simulink model "Full_Car_Model"  (R2023b)
settings: Solver=FixedStepAuto  StartTime=0.0  StopTime=t_end_sim  FixedStep=Ts_sim  RelTol=1e-3
values from neighbouring files (symbols this model uses):
  a_b_ref_sat = [ zeros(1,10) ... (first row only)    [A1_Init.m]    (also in C1_MonteCarloAnalysis.m)
  adaptive = 3    [A1_Init.m]    (also in C1_MonteCarloAnalysis.m = 1)
  data = A2_Full_car_model_parameters_4onBoard()    [A1_Init.m]    (also in C1_MonteCarloAnalysis.m)
  Ft_demand_F = [zeros(1,601) 200*ones(1,2400)]./data.R_F    [A1_Init.m]    (also in C1_MonteCarloAnalysis.m)
  Ft_demand_R = [zeros(1,(601-length(l_discr)))              200*ones(1,(2400+length(l_discr)))]./data.R_R    [A1_Init.m]    (also in C1_MonteCarloAnalysis.m)
  handmade_front = strcat(currentPath,'\Road_profiles\height_crg_files\','handmade_step_3cm_singlefunctions.crg')    [A1_Init.m]    (also in C1_MonteCarloAnalysis.m)
  handmade_mu_front = strcat(currentPath,'\Road_profiles\friction_crg_files\','handmade_fric_step_01_singlefunctions.crg')    [A1_Init.m]    (also in C1_MonteCarloAnalysis.m)
  handmade_mu_rear = handmade_mu_front    [A1_Init.m]    (also in C1_MonteCarloAnalysis.m)
  handmade_rear = handmade_front    [A1_Init.m]    (also in C1_MonteCarloAnalysis.m)
  LowLim_Q1 = -10    [A1_Init.m]    (also in C1_MonteCarloAnalysis.m)
  M = N    (= 10)    [A1_Init.m]    (also in C1_MonteCarloAnalysis.m)
  mu_distance = test_distance    [A1_Init.m]    (also in C1_MonteCarloAnalysis.m)
  mu_road = [ones(1,1001), 0.1*ones(1,2000)]    [A1_Init.m]    (also in C1_MonteCarloAnalysis.m)
  N = 10    [A1_Init.m]    (also in C1_MonteCarloAnalysis.m)
  N_iter = 3    [A1_Init.m]    (also in C1_MonteCarloAnalysis.m)
  omega_ini_F_L = x_u_dot_ini_F_L/data.R_F    [A1_Init.m]    (also in C1_MonteCarloAnalysis.m)
  omega_ini_F_R = x_u_dot_ini_R_R/data.R_F    [A1_Init.m]    (also in C1_MonteCarloAnalysis.m)
  omega_ini_R_L = x_u_dot_ini_R_L/data.R_R +2.483*1e-6    [A1_Init.m]    (also in C1_MonteCarloAnalysis.m)
  omega_ini_R_R = x_u_dot_ini_R_R/data.R_R+2.483*1e-6    [A1_Init.m]    (also in C1_MonteCarloAnalysis.m)
  passive = 2    [A1_Init.m]    (also in C1_MonteCarloAnalysis.m)
  Pitch = 0    [A1_Init.m]    (also in C1_MonteCarloAnalysis.m)
  Pitch_dot = 0    [A1_Init.m]    (also in C1_MonteCarloAnalysis.m)
  preview = 2    [A1_Init.m]    (also in C1_MonteCarloAnalysis.m)
  Q1 = 1e6    (= 1000000)    [A1_Init.m]    (also in C1_MonteCarloAnalysis.m)
  Q1_sat = 0    [A1_Init.m]    (also in C1_MonteCarloAnalysis.m)
  Q2 = 1e5    (= 100000)    [A1_Init.m]    (also in C1_MonteCarloAnalysis.m)
  QN1 = 0    [A1_Init.m]    (also in C1_MonteCarloAnalysis.m)
  QN2 = 0    [A1_Init.m]    (also in C1_MonteCarloAnalysis.m)
  R1 = 1e10    (= 10000000000)    [A1_Init.m]    (also in C1_MonteCarloAnalysis.m)
  r1_h0 = 0.99    [A1_Init.m]    (also in C1_MonteCarloAnalysis.m)
  r1_k = 1000    [A1_Init.m]    (also in C1_MonteCarloAnalysis.m)
  r1_max = 11    [A1_Init.m]    (also in C1_MonteCarloAnalysis.m)
  r1_min = -10    [A1_Init.m]    (also in C1_MonteCarloAnalysis.m)
  r2 = 2    [A1_Init.m]    (also in C1_MonteCarloAnalysis.m)
  R2 = 1e2    (= 100)    [A1_Init.m]    (also in C1_MonteCarloAnalysis.m)
  R2_rl = 2    [A1_Init.m]    (also in C1_MonteCarloAnalysis.m)
  road_profile = [zeros(1,801),ones(1,2200)*10*Step_selector]    [A1_Init.m]    (also in C1_MonteCarloAnalysis.m)
  T_distance = test_distance    [A1_Init.m]    (also in C1_MonteCarloAnalysis.m)
  T_hs_ini_F_L = 0    [A1_Init.m]    (also in C1_MonteCarloAnalysis.m)
  T_hs_ini_F_R = 0    [A1_Init.m]    (also in C1_MonteCarloAnalysis.m)
  T_hs_ini_R_L = 0    [A1_Init.m]    (also in C1_MonteCarloAnalysis.m)
  T_hs_ini_R_R = 0    [A1_Init.m]    (also in C1_MonteCarloAnalysis.m)
  test_distance = 0:0.01:30    [A1_Init.m]    (also in C1_MonteCarloAnalysis.m)
  theta_s_ini_F_L = 0    [A1_Init.m]    (also in C1_MonteCarloAnalysis.m)
  theta_s_ini_F_R = 0    [A1_Init.m]    (also in C1_MonteCarloAnalysis.m)
  theta_s_ini_R_L = 0    [A1_Init.m]    (also in C1_MonteCarloAnalysis.m)
  theta_s_ini_R_R = 0    [A1_Init.m]    (also in C1_MonteCarloAnalysis.m)
  theta_w_ini_F_L = -1.056*1e-2    (= -0.01056)    [A1_Init.m]    (also in C1_MonteCarloAnalysis.m)
  theta_w_ini_R_L = -1.056*1e-2    (= -0.01056)    [A1_Init.m]    (also in C1_MonteCarloAnalysis.m)
  Ts = 1e-3*[0 5 10 15 20 25 30 40 60 80 100]    [A1_Init.m]    (also in C1_MonteCarloAnalysis.m)
  w1_h0 = 0.0008    [A1_Init.m]    (also in C1_MonteCarloAnalysis.m)
  w1_k = 5000    [A1_Init.m]    (also in C1_MonteCarloAnalysis.m)
  w1_max = 9    [A1_Init.m]    (also in C1_MonteCarloAnalysis.m)
  w1_min = -10    [A1_Init.m]    (also in C1_MonteCarloAnalysis.m)
  w1_sat = 0.085    [A1_Init.m]    (also in C1_MonteCarloAnalysis.m)
  w2_h0 = 2    [A1_Init.m]    (also in C1_MonteCarloAnalysis.m)
  w2_inc = 0.05    [A1_Init.m]    (also in C1_MonteCarloAnalysis.m)
  w2_k = 10    [A1_Init.m]    (also in C1_MonteCarloAnalysis.m)
  w2_max = 5.3    [A1_Init.m]    (also in C1_MonteCarloAnalysis.m)
  w2_min = -10    [A1_Init.m]    (also in C1_MonteCarloAnalysis.m)
  Wmat_NMPC_init = [W(1,:) W(2,:) W(3,:) W(4,:)]    [A1_Init.m]    (also in C1_MonteCarloAnalysis.m)
  WNmat_NMPC_init = [WN(1,:) WN(2,:)]    [A1_Init.m]    (also in C1_MonteCarloAnalysis.m)
  X_0 = [z_b_dot_ini z_b_ini z_u_dot_ini_F_L z_u_ini_F_L x_b_dot_ini x_b_ini x_u_dot_ini_F_L x_u_ini_F_L          omega_ini_F_L theta_w_ini_F_L omega_ini_F_L theta_s_ini_F_L torque_ini_F_L]    [A1_Init.m]    (also in C1_MonteCarloAnalysis.m)
  x_b_dot_ini = speed_ini/3.6    (= 11.1111111111)    [A1_Init.m]    (also in C1_MonteCarloAnalysis.m)
  x_b_ini = data.b+pos_ini    [A1_Init.m]    (also in C1_MonteCarloAnalysis.m)
  x_u_dot_ini_F_L = speed_ini/3.6 - 1.125*1e-4    (= 11.1109986111)    [A1_Init.m]    (also in C1_MonteCarloAnalysis.m)
  x_u_dot_ini_F_R = speed_ini/3.6 - 1.125*1e-4    (= 11.1109986111)    [A1_Init.m]    (also in C1_MonteCarloAnalysis.m)
  x_u_dot_ini_R_L = speed_ini/3.6 - 1.125*1e-4    (= 11.1109986111)    [A1_Init.m]    (also in C1_MonteCarloAnalysis.m)
  x_u_dot_ini_R_R = speed_ini/3.6 - 1.125*1e-4    (= 11.1109986111)    [A1_Init.m]    (also in C1_MonteCarloAnalysis.m)
  x_u_ini_F_L = data.a+data.b+pos_ini    [A1_Init.m]    (also in C1_MonteCarloAnalysis.m)
  x_u_ini_F_R = data.a+data.b+pos_ini    [A1_Init.m]    (also in C1_MonteCarloAnalysis.m)
  x_u_ini_R_L = pos_ini    (= 0)    [A1_Init.m]    (also in C1_MonteCarloAnalysis.m)
  x_u_ini_R_R = pos_ini    (= 0)    [A1_Init.m]    (also in C1_MonteCarloAnalysis.m)
  z_b_dot_ini = 0    [A1_Init.m]    (also in C1_MonteCarloAnalysis.m)
  z_b_ini = 0    [A1_Init.m]    (also in C1_MonteCarloAnalysis.m)
  z_u_dot_ini_F_L = 0    [A1_Init.m]    (also in C1_MonteCarloAnalysis.m)
  z_u_dot_ini_F_R = 0    [A1_Init.m]    (also in C1_MonteCarloAnalysis.m)
  z_u_dot_ini_R_L = 0    [A1_Init.m]    (also in C1_MonteCarloAnalysis.m)
  z_u_dot_ini_R_R = 0    [A1_Init.m]    (also in C1_MonteCarloAnalysis.m)
  z_u_ini_F_L = 0    [A1_Init.m]    (also in C1_MonteCarloAnalysis.m)
  z_u_ini_F_R = 0    [A1_Init.m]    (also in C1_MonteCarloAnalysis.m)
  z_u_ini_R_L = 0    [A1_Init.m]    (also in C1_MonteCarloAnalysis.m)
  z_u_ini_R_R = 0    [A1_Init.m]    (also in C1_MonteCarloAnalysis.m)
undefined symbols (not defined in the file or in its folder): Delay_step, road_with_noise
libraries: mfswift_library x8, rllib x4, simulink x4
(part 5 of 7)

== system Full_Car_Model/CONTROLLER REAR RIGHT/Rule based/Subsystem ==
  Online Data : Inport
  Delay{,1..4} (5 alike) : Delay  DelayLength=10
  Delay{5..34} (30 alike) : Delay  DelayLength=1
  MATLAB Function : MATLAB Function  TreatAsAtomicUnit=on
  Mux : Mux  Inputs=5
  Mux1 : Mux  Inputs=30
  Mux2 : Mux  Inputs=2
  Rate Transition : RateTransition  OutPortSampleTime=Ts(2)
  Rate Transition1 : RateTransition  OutPortSampleTime=Ts(2)
  Selector : Selector  NumberOfDimensions=2  InputPortWidth=1  IndexOptions=Index vector (dialog),Select all  Indices=1,1  OutputSizes=1,1
  Selector1 : Selector  NumberOfDimensions=2  InputPortWidth=1  IndexOptions=Index vector (dialog),Select all  Indices=1,1  OutputSizes=1,1
  w_prev : Outport
  mu_act_prev : Outport  Port=2
  wires:
  MATLAB Function/1(w) -> Mux2/2, Selector/1, Selector1/1
  MATLAB Function/2(mu_act) -> mu_act_prev/1
  Mux1/1 -> Rate Transition1/1
  Rate Transition/1 -> MATLAB Function/1(OnlineData)
  Mux2/1 -> w_prev/1
  Delay4/1 -> Mux/1
  Delay3/1 -> Delay4/1, Mux/2
  Delay2/1 -> Delay3/1, Mux/3
  Delay1/1 -> Mux/4, Delay2/1
  Delay/1 -> Mux/5, Delay1/1
  Selector/1 -> Delay/1  "w1"
  Online Data/1 -> Rate Transition/1
  Delay5/1 -> Mux1/8, Delay10/1
  Selector1/1 -> Delay29/1  "w1"
  Delay10/1 -> Mux1/7, Delay11/1
  Delay11/1 -> Mux1/6, Delay12/1
  Delay12/1 -> Mux1/5, Delay13/1
  Delay13/1 -> Mux1/4, Delay14/1
  Delay14/1 -> Mux1/3, Delay15/1
  Delay15/1 -> Mux1/2, Delay16/1
  Delay16/1 -> Mux1/1
  Delay6/1 -> Mux1/9, Delay5/1
  Delay7/1 -> Mux1/10, Delay6/1
  Delay8/1 -> Delay7/1, Mux1/11
  Delay9/1 -> Mux1/12, Delay8/1
  Delay17/1 -> Mux1/13, Delay9/1
  Delay18/1 -> Mux1/14, Delay17/1
  Delay19/1 -> Delay18/1, Mux1/15
  Delay26/1 -> Mux1/16, Delay19/1
  Delay25/1 -> Mux1/17, Delay26/1
  Delay24/1 -> Mux1/18, Delay25/1
  Delay22/1 -> Mux1/20, Delay23/1
  Delay34/1 -> Mux1/27, Delay33/1
  Delay33/1 -> Mux1/26, Delay32/1
  Delay31/1 -> Mux1/24, Delay30/1
  Delay32/1 -> Mux1/25, Delay31/1
  Delay30/1 -> Mux1/23, Delay20/1
  Delay28/1 -> Mux1/29, Delay27/1
  Delay27/1 -> Mux1/28, Delay34/1
  Delay23/1 -> Mux1/19, Delay24/1
  Delay21/1 -> Mux1/21, Delay22/1
  Delay29/1 -> Mux1/30, Delay28/1
  Delay20/1 -> Mux1/22, Delay21/1
  Mux/1 -> Mux2/1

== system Full_Car_Model/CONTROLLER REAR RIGHT/Rule based/memory ==
  In1 : Inport
  Abs : Abs  SaturateOnIntegerOverflow=off
  Add : Sum  Inputs=-+
  Memory{,1..10,12..15,19,26..49} (40 alike) : Memory  InheritSampleTime=on
  Mux1 : Mux  Inputs=40
  Rate Transition : RateTransition  OutPortSampleTime=Ts(2)
  Out1 : Outport
  wires:
  Abs/1 -> Mux1/40, Memory49/1
  Memory49/1 -> Mux1/39, Memory19/1
  Memory19/1 -> Memory35/1, Mux1/38
  Memory47/1 -> Memory48/1, Mux1/31
  Memory42/1 -> Memory43/1, Mux1/36
  Memory44/1 -> Memory45/1, Mux1/34
  Memory43/1 -> Memory44/1, Mux1/35
  Memory33/1 -> Memory34/1, Mux1/23
  Memory46/1 -> Memory47/1, Mux1/32
  Memory32/1 -> Memory33/1, Mux1/24
  Memory38/1 -> Memory39/1, Mux1/18
  Memory48/1 -> Memory26/1, Mux1/30
  Memory45/1 -> Memory46/1, Mux1/33
  Memory30/1 -> Memory31/1, Mux1/26
  Memory26/1 -> Memory28/1, Mux1/29
  Memory37/1 -> Memory38/1, Mux1/19
  Memory29/1 -> Memory30/1, Mux1/27
  Memory31/1 -> Memory32/1, Mux1/25
  Memory27/1 -> Memory36/1, Mux1/21
  Memory28/1 -> Memory29/1, Mux1/28
  Memory34/1 -> Memory27/1, Mux1/22
  Memory40/1 -> Memory41/1, Mux1/16
  Memory41/1 -> Mux1/15, Memory1/1
  Memory39/1 -> Memory40/1, Mux1/17
  Memory35/1 -> Memory42/1, Mux1/37
  Memory36/1 -> Memory37/1, Mux1/20
  Add/1 -> Abs/1
  In1/1 -> Rate Transition/1
  Memory/1 -> Add/1
  Rate Transition/1 -> Add/2, Memory/1
  Memory14/1 -> Memory15/1, Mux1/2
  Memory12/1 -> Memory13/1, Mux1/4
  Memory15/1 -> Mux1/1
  Memory13/1 -> Memory14/1, Mux1/3
  Memory10/1 -> Mux1/5, Memory12/1
  Memory9/1 -> Memory10/1, Mux1/6
  Memory8/1 -> Memory9/1, Mux1/7
  Memory7/1 -> Memory8/1, Mux1/8
  Memory6/1 -> Memory7/1, Mux1/9
  Memory5/1 -> Memory6/1, Mux1/10
  Memory4/1 -> Mux1/11, Memory5/1
  Memory3/1 -> Memory4/1, Mux1/12
  Memory2/1 -> Mux1/13, Memory3/1
  Memory1/1 -> Memory2/1, Mux1/14
  Mux1/1 -> Out1/1

== system Full_Car_Model/PLANT MODEL WITH MF-SWIFT/4 ON-BOARD POWERTRAIN - FRONT/DIFFERENTIAL_L ==
  T_dm : Inport
  Multiply : Gain  Gain=data.i_g1_F4
  Multiply1 : Gain  Gain=data.n_g1_F4
  Multiply2 : Gain  Gain=data.i_g2_F4
  Multiply3 : Gain  Gain=data.n_g2_F4
  T_t : Outport
  wires:
  T_dm/1 -> Multiply/1
  Multiply3/1 -> T_t/1
  Multiply1/1 -> Multiply2/1
  Multiply2/1 -> Multiply3/1
  Multiply/1 -> Multiply1/1

== system Full_Car_Model/PLANT MODEL WITH MF-SWIFT/4 ON-BOARD POWERTRAIN - FRONT/DIFFERENTIAL_R ==
  T_dm : Inport
  Multiply : Gain  Gain=data.i_g1_F4
  Multiply1 : Gain  Gain=data.n_g1_F4
  Multiply2 : Gain  Gain=data.i_g2_F4
  Multiply3 : Gain  Gain=data.n_g2_F4
  T_t : Outport
  wires:
  Multiply3/1 -> T_t/1
  Multiply/1 -> Multiply1/1
  Multiply1/1 -> Multiply2/1
  Multiply2/1 -> Multiply3/1
  T_dm/1 -> Multiply/1

== system Full_Car_Model/PLANT MODEL WITH MF-SWIFT/4 ON-BOARD POWERTRAIN - FRONT/LEFT HALF SHAFT TORQUES WITH BACKLASH ==
  omega_s : Inport
  theta_s : Inport  Port=2
  theta_w : Inport  Port=3
  omega_w : Inport  Port=4
  Add1 : Sum  Inputs=+-
  Add2 : Sum  Inputs=+-
  Add{3..5,7} (4 alike) : Sum
  Add6 : Sum  Inputs=+-
  Constant : Constant  Value=data.backlash_F4
  Constant1 : Constant  Value=data.backlash_F4
  Constant2 : Constant  Value=data.backlash_F4
  MATLAB Function2 : MATLAB Function  TreatAsAtomicUnit=on
  MATLAB Function3 : MATLAB Function  TreatAsAtomicUnit=on
  Multiply1 : Gain  Gain=data.k_hs_F4
  Multiply2 : Gain  Gain=data.k_hs_F4
  Multiply3 : Gain  Gain=data.b_hs_F4
  Product{1..4} (4 alike) : Product
  T_hs : Outport
  wires:
  [delta_omega_F_L] -> Multiply3/1
  [delta_theta_F_L] -> MATLAB Function3/1(delta_theta)
  Add1/1 -> [delta_omega_F_L]  "delta_omega"
  [delta_theta_F_L] -> Add6/1
  [delta_theta_F_L] -> Add7/1
  [delta_theta_F_L] -> MATLAB Function2/1(delta_theta)
  Add2/1 -> [delta_theta_F_L]  "delta_theta"
  Multiply3/1 -> Product4/1, Product3/1  "fc"
  Add6/1 -> Multiply1/1
  Constant1/1 -> Add6/2
  Multiply1/1 -> Product1/1  "fb"
  Constant/1 -> Add7/2
  Add7/1 -> Multiply2/1
  Product1/1 -> Add4/2
  Product2/1 -> Add4/1
  Product3/1 -> Add3/1
  Product4/1 -> Add3/2
  Add3/1 -> Add5/2  "T_hs_D"
  Add4/1 -> Add5/1  "T_hs_S"
  MATLAB Function3/1(f2) -> Product4/2, Product1/2  "f2"
  MATLAB Function2/1(f1) -> Product3/2, Product2/2  "f1"
  Multiply2/1 -> Product2/1  "fa"
  omega_s/1 -> Add1/1
  omega_w/1 -> Add1/2
  theta_w/1 -> Add2/2
  theta_s/1 -> Add2/1
  Add5/1 -> T_hs/1
  Constant2/1 -> MATLAB Function2/2(backlash_F4), MATLAB Function3/2(backlash_F4)

== system Full_Car_Model/PLANT MODEL WITH MF-SWIFT/4 ON-BOARD POWERTRAIN - FRONT/RIGHT HALF SHAFT TORQUES WITH BACKLASH ==
  omega_s : Inport
  theta_s : Inport  Port=2
  theta_w : Inport  Port=3
  omega_w : Inport  Port=4
  Add1 : Sum  Inputs=+-
  Add2 : Sum  Inputs=+-
  Add{3..5,7} (4 alike) : Sum
  Add6 : Sum  Inputs=+-
  Constant : Constant  Value=data.backlash_F4
  Constant1 : Constant  Value=data.backlash_F4
  Constant2 : Constant  Value=data.backlash_F4
  MATLAB Function2 : MATLAB Function  TreatAsAtomicUnit=on
  MATLAB Function3 : MATLAB Function  TreatAsAtomicUnit=on
  Multiply1 : Gain  Gain=data.k_hs_F4
  Multiply2 : Gain  Gain=data.k_hs_F4
  Multiply3 : Gain  Gain=data.b_hs_F4
  Product{1..4} (4 alike) : Product
  T_hs : Outport
  wires:
  Add5/1 -> T_hs/1
  theta_s/1 -> Add2/1
  theta_w/1 -> Add2/2
  omega_w/1 -> Add1/2
  omega_s/1 -> Add1/1
  Multiply2/1 -> Product2/1  "fa"
  MATLAB Function2/1(f1) -> Product3/2, Product2/2  "f1"
  MATLAB Function3/1(f2) -> Product1/2, Product4/2  "f2"
  Add4/1 -> Add5/1  "T_hs_S"
  Add3/1 -> Add5/2  "T_hs_D"
  Product4/1 -> Add3/2
  Product3/1 -> Add3/1
  Product2/1 -> Add4/1
  Product1/1 -> Add4/2
  Add7/1 -> Multiply2/1
  Constant/1 -> Add7/2
  Multiply1/1 -> Product1/1  "fb"
  Constant1/1 -> Add6/2
  Add6/1 -> Multiply1/1
  Multiply3/1 -> Product3/1, Product4/1  "fc"
  Add2/1 -> [delta_theta_F_R]  "delta_theta"
  [delta_theta_F_R] -> MATLAB Function2/1(delta_theta)
  [delta_theta_F_R] -> Add7/1
  [delta_theta_F_R] -> Add6/1
  Add1/1 -> [delta_omega_F_R]  "delta_omega"
  [delta_theta_F_R] -> MATLAB Function3/1(delta_theta)
  [delta_omega_F_R] -> Multiply3/1
  Constant2/1 -> MATLAB Function3/2(backlash_F4), MATLAB Function2/2(backlash_F4)

== system Full_Car_Model/PLANT MODEL WITH MF-SWIFT/4 ON-BOARD POWERTRAIN - REAR/DIFFERENTIAL_L ==
  T_dm : Inport
  Multiply : Gain  Gain=data.i_g1_R4
  Multiply1 : Gain  Gain=data.n_g1_R4
  Multiply2 : Gain  Gain=data.i_g2_R4
  Multiply3 : Gain  Gain=data.n_g2_R4
  T_t : Outport
  wires:
  T_dm/1 -> Multiply/1
  Multiply3/1 -> T_t/1
  Multiply1/1 -> Multiply2/1
  Multiply2/1 -> Multiply3/1
  Multiply/1 -> Multiply1/1

== system Full_Car_Model/PLANT MODEL WITH MF-SWIFT/4 ON-BOARD POWERTRAIN - REAR/DIFFERENTIAL_R ==
  T_dm : Inport
  Multiply : Gain  Gain=data.i_g1_R4
  Multiply1 : Gain  Gain=data.n_g1_R4
  Multiply2 : Gain  Gain=data.i_g2_R4
  Multiply3 : Gain  Gain=data.n_g2_R4
  T_t : Outport
  wires:
  Multiply/1 -> Multiply1/1
  Multiply2/1 -> Multiply3/1
  Multiply1/1 -> Multiply2/1
  Multiply3/1 -> T_t/1
  T_dm/1 -> Multiply/1

== system Full_Car_Model/PLANT MODEL WITH MF-SWIFT/4 ON-BOARD POWERTRAIN - REAR/LEFT HALF SHAFT TORQUES WITH BACKLASH ==
  omega_s : Inport
  theta_s : Inport  Port=2
  theta_w : Inport  Port=3
  omega_w : Inport  Port=4
  Add1 : Sum  Inputs=+-
  Add2 : Sum  Inputs=+-
  Add{3..5,7} (4 alike) : Sum
  Add6 : Sum  Inputs=+-
  Constant : Constant  Value=data.backlash_R4
  Constant1 : Constant  Value=data.backlash_R4
  Constant2 : Constant  Value=data.backlash_R4
  MATLAB Function2 : MATLAB Function  TreatAsAtomicUnit=on
  MATLAB Function3 : MATLAB Function  TreatAsAtomicUnit=on
  Multiply1 : Gain  Gain=data.k_hs_R4
  Multiply2 : Gain  Gain=data.k_hs_R4
  Multiply3 : Gain  Gain=data.b_hs_R4
  Product{1..4} (4 alike) : Product
  T_hs : Outport
  wires:
  [delta_omega_R_L] -> Multiply3/1
  [delta_theta_R_L] -> MATLAB Function3/1(delta_theta)
  Add1/1 -> [delta_omega_R_L]  "delta_omega"
  [delta_theta_R_L] -> Add6/1
  [delta_theta_R_L] -> Add7/1
  [delta_theta_R_L] -> MATLAB Function2/1(delta_theta)
  Add2/1 -> [delta_theta_R_L]  "delta_theta"
  Multiply3/1 -> Product4/1, Product3/1  "fc"
  Add6/1 -> Multiply1/1
  Constant1/1 -> Add6/2
  Multiply1/1 -> Product1/1  "fb"
  Constant/1 -> Add7/2
  Add7/1 -> Multiply2/1
  Product1/1 -> Add4/2
  Product2/1 -> Add4/1
  Product3/1 -> Add3/1
  Product4/1 -> Add3/2
  Add3/1 -> Add5/2  "T_hs_D"
  Add4/1 -> Add5/1  "T_hs_S"
  MATLAB Function3/1(f2) -> Product4/2, Product1/2  "f2"
  MATLAB Function2/1(f1) -> Product3/2, Product2/2  "f1"
  Multiply2/1 -> Product2/1  "fa"
  omega_s/1 -> Add1/1
  omega_w/1 -> Add1/2
  theta_w/1 -> Add2/2
  theta_s/1 -> Add2/1
  Add5/1 -> T_hs/1
  Constant2/1 -> MATLAB Function3/2(backlash_R4), MATLAB Function2/2(backlash_R4)

== system Full_Car_Model/PLANT MODEL WITH MF-SWIFT/4 ON-BOARD POWERTRAIN - REAR/RIGHT HALF SHAFT TORQUES WITH BACKLASH ==
  omega_s : Inport
  theta_s : Inport  Port=2
  theta_w : Inport  Port=3
  omega_w : Inport  Port=4
  Add1 : Sum  Inputs=+-
  Add2 : Sum  Inputs=+-
  Add{3..5,7} (4 alike) : Sum
  Add6 : Sum  Inputs=+-
  Constant : Constant  Value=data.backlash_R4
  Constant1 : Constant  Value=data.backlash_R4
  Constant2 : Constant  Value=data.backlash_R4
  MATLAB Function2 : MATLAB Function  TreatAsAtomicUnit=on
  MATLAB Function3 : MATLAB Function  TreatAsAtomicUnit=on
  Multiply1 : Gain  Gain=data.k_hs_R4
  Multiply2 : Gain  Gain=data.k_hs_R4
  Multiply3 : Gain  Gain=data.b_hs_R4
  Product{1..4} (4 alike) : Product
  T_hs : Outport
  wires:
  Add5/1 -> T_hs/1
  theta_s/1 -> Add2/1
  theta_w/1 -> Add2/2
  omega_w/1 -> Add1/2
  omega_s/1 -> Add1/1
  Multiply2/1 -> Product2/1  "fa"
  MATLAB Function2/1(f1) -> Product3/2, Product2/2  "f1"
  MATLAB Function3/1(f2) -> Product1/2, Product4/2  "f2"
  Add4/1 -> Add5/1  "T_hs_S"
  Add3/1 -> Add5/2  "T_hs_D"
  Product4/1 -> Add3/2
  Product3/1 -> Add3/1
  Product2/1 -> Add4/1
  Product1/1 -> Add4/2
  Add7/1 -> Multiply2/1
  Constant/1 -> Add7/2
  Multiply1/1 -> Product1/1  "fb"
  Constant1/1 -> Add6/2
  Add6/1 -> Multiply1/1
  Multiply3/1 -> Product3/1, Product4/1  "fc"
  Add2/1 -> [delta_theta_R_R]  "delta_theta"
  [delta_theta_R_R] -> MATLAB Function2/1(delta_theta)
  [delta_theta_R_R] -> Add7/1
  [delta_theta_R_R] -> Add6/1
  Add1/1 -> [delta_omega_R_R]  "delta_omega"
  [delta_theta_R_R] -> MATLAB Function3/1(delta_theta)
  [delta_omega_R_R] -> Multiply3/1
  Constant2/1 -> MATLAB Function3/2(backlash_R4), MATLAB Function2/2(backlash_R4)

== system Full_Car_Model/PLANT MODEL WITH MF-SWIFT/FRONT LEFT WHEEL/Subsystem ==
  speed : Inport
  Bus Selector : BusSelector  OutputSignals=States.x_u_dot_F_L,States.z_u_dot_F_L
  Constant : Constant  Value=0
  Mux : Mux  Inputs=3
  Velocity : Outport  VectorParamsAs1DForOutWhenUnconnected=off
  wires:
  Bus Selector/2 -> Mux/3  "<z_u_dot_F_L>"
  Bus Selector/1 -> Mux/1  "<x_u_dot_F_L>"
  speed/1 -> Bus Selector/1
  Mux/1 -> Velocity/1
  Constant/1 -> Mux/2  "No lateral component"

== system Full_Car_Model/PLANT MODEL WITH MF-SWIFT/FRONT LEFT WHEEL/Subsystem1 ==
  Angular Speed : Inport
  Constant1 : Constant  Value=0
  Constant2 : Constant  Value=0
  Constant3 : Constant  Value=0
  Mux : Mux  Inputs=3
  Terminator : Terminator
  AngularVelocity : Outport  VectorParamsAs1DForOutWhenUnconnected=off
  wires:
  Constant3/1 -> Mux/2
  Constant1/1 -> Mux/3
  Constant2/1 -> Mux/1
  Angular Speed/1 -> Terminator/1
  Mux/1 -> AngularVelocity/1

== system Full_Car_Model/PLANT MODEL WITH MF-SWIFT/FRONT LEFT WHEEL/Subsystem6 ==
  time : Inport
  gain : Inport  Port=2
  Demux : Demux  Outputs=9
  Multiply : Product  Inputs=**
  Mux : Mux  Inputs=20
  Step : Step  After=0.02  SampleTime=0
  Terminator : Terminator
  ground{,1..7} (8 alike) : Ground
  rotation matrix : Constant  Value=[1 0 0 0 1 0 0 0 1]
  surface friction in lateral direction : Constant
  surface friction in longitudinall direction : Constant
  Road : Outport  VectorParamsAs1DForOutWhenUnconnected=off
  wires:
  Multiply/1 -> Mux/3
  Step/1 -> Multiply/1
  gain/1 -> Multiply/2
  time/1 -> Terminator/1
  Demux/9 -> Mux/12
  Demux/8 -> Mux/11
  Demux/7 -> Mux/10
  Demux/6 -> Mux/9
  Demux/5 -> Mux/8
  Demux/4 -> Mux/7
  Demux/3 -> Mux/6
  Demux/2 -> Mux/5
  Demux/1 -> Mux/4
  rotation matrix/1 -> Demux/1
  surface friction in lateral direction/1 -> Mux/20
  surface friction in longitudinall direction/1 -> Mux/19
  ground7/1 -> Mux/18
  ground6/1 -> Mux/17
  ground5/1 -> Mux/16
  ground4/1 -> Mux/15
  ground3/1 -> Mux/14
  ground2/1 -> Mux/13
  ground1/1 -> Mux/2
  ground/1 -> Mux/1
  Mux/1 -> Road/1

== system Full_Car_Model/PLANT MODEL WITH MF-SWIFT/FRONT RIGHT WHEEL/Subsystem ==
  speed : Inport
  Bus Selector : BusSelector  OutputSignals=States.x_u_dot_F_R,States.z_u_dot_F_R
  Constant : Constant  Value=0
  Mux : Mux  Inputs=3
  Velocity : Outport  VectorParamsAs1DForOutWhenUnconnected=off
  wires:
  Constant/1 -> Mux/2  "No lateral component"
  Mux/1 -> Velocity/1
  speed/1 -> Bus Selector/1
  Bus Selector/1 -> Mux/1  "<x_u_dot_F_R>"
  Bus Selector/2 -> Mux/3  "<z_u_dot_F_R>"

== system Full_Car_Model/PLANT MODEL WITH MF-SWIFT/FRONT RIGHT WHEEL/Subsystem1 ==
  Angular Speed : Inport
  Constant1 : Constant  Value=0
  Constant2 : Constant  Value=0
  Constant3 : Constant  Value=0
  Mux : Mux  Inputs=3
  Terminator : Terminator
  AngularVelocity : Outport  VectorParamsAs1DForOutWhenUnconnected=off
  wires:
  Mux/1 -> AngularVelocity/1
  Angular Speed/1 -> Terminator/1
  Constant2/1 -> Mux/1
  Constant1/1 -> Mux/3
  Constant3/1 -> Mux/2

== system Full_Car_Model/PLANT MODEL WITH MF-SWIFT/FRONT RIGHT WHEEL/Subsystem6 ==
  time : Inport
  gain : Inport  Port=2
  Demux : Demux  Outputs=9
  Multiply : Product  Inputs=**
  Mux : Mux  Inputs=20
  Step : Step  After=0.02  SampleTime=0
  Terminator : Terminator
  ground{,1..7} (8 alike) : Ground
  rotation matrix : Constant  Value=[1 0 0 0 1 0 0 0 1]
  surface friction in lateral direction : Constant
  surface friction in longitudinall direction : Constant
  Road : Outport  VectorParamsAs1DForOutWhenUnconnected=off
  wires:
  Mux/1 -> Road/1
  ground/1 -> Mux/1
  ground1/1 -> Mux/2
  ground2/1 -> Mux/13
  ground3/1 -> Mux/14
  ground4/1 -> Mux/15
  ground5/1 -> Mux/16
  ground6/1 -> Mux/17
  ground7/1 -> Mux/18
  surface friction in longitudinall direction/1 -> Mux/19
  surface friction in lateral direction/1 -> Mux/20
  rotation matrix/1 -> Demux/1
  Demux/1 -> Mux/4
  Demux/2 -> Mux/5
  Demux/3 -> Mux/6
  Demux/4 -> Mux/7
  Demux/5 -> Mux/8
  Demux/6 -> Mux/9
  Demux/7 -> Mux/10
  Demux/8 -> Mux/11
  Demux/9 -> Mux/12
  time/1 -> Terminator/1
  gain/1 -> Multiply/2
  Step/1 -> Multiply/1
  Multiply/1 -> Mux/3

== system Full_Car_Model/PLANT MODEL WITH MF-SWIFT/REAR LEFT WHEEL/Subsystem2 ==
  speed : Inport
  Bus Selector : BusSelector  OutputSignals=States.x_u_dot_R_L,States.z_u_dot_R_L
  Constant : Constant  Value=0
  Mux : Mux  Inputs=3
  Velocity : Outport  VectorParamsAs1DForOutWhenUnconnected=off
  wires:
  Bus Selector/2 -> Mux/3  "<z_u_dot_R_L>"
  speed/1 -> Bus Selector/1
  Mux/1 -> Velocity/1
  Constant/1 -> Mux/2  "No lateral component"
  Bus Selector/1 -> Mux/1  "<x_u_dot_R_L>"

== system Full_Car_Model/PLANT MODEL WITH MF-SWIFT/REAR LEFT WHEEL/Subsystem5 ==
  Angular Speed : Inport
  Constant1 : Constant  Value=0
  Constant2 : Constant  Value=0
  Constant3 : Constant  Value=0
  Mux : Mux  Inputs=3
  Terminator : Terminator
  AngularVelocity : Outport  VectorParamsAs1DForOutWhenUnconnected=off
  wires:
  Constant1/1 -> Mux/3
  Constant2/1 -> Mux/1
  Angular Speed/1 -> Terminator/1
  Mux/1 -> AngularVelocity/1
  Constant3/1 -> Mux/2

== system Full_Car_Model/PLANT MODEL WITH MF-SWIFT/REAR LEFT WHEEL/Subsystem7 ==
  time : Inport
  gain : Inport  Port=2
  Demux1 : Demux  Outputs=9
  Multiply : Product  Inputs=**
  Mux1 : Mux  Inputs=20
  Step : Step  Time=1.216  After=0.02  SampleTime=0
  Terminator : Terminator
  ground{,1..7} (8 alike) : Ground
  rotation matrix1 : Constant  Value=[1 0 0 0 1 0 0 0 1]
  surface friction in lateral direction : Constant
  surface friction in lateral direction1 : Constant
  surface friction in longitudinall direction : Constant
  Road : Outport  VectorParamsAs1DForOutWhenUnconnected=off
  wires:
  time/1 -> Terminator/1
  Demux1/4 -> Mux1/7
  Multiply/1 -> Mux1/3
  Demux1/5 -> Mux1/8
  rotation matrix1/1 -> Demux1/1
  surface friction in lateral direction/1 -> Mux1/20
  ground2/1 -> Mux1/13
  Demux1/2 -> Mux1/5
  ground7/1 -> Mux1/18
  ground6/1 -> Mux1/17
  Demux1/3 -> Mux1/6
  ground1/1 -> Mux1/2
  Step/1 -> Multiply/1
  Demux1/7 -> Mux1/10
  Demux1/8 -> Mux1/11
  ground/1 -> Mux1/1
  Demux1/6 -> Mux1/9
  ground5/1 -> Mux1/16
  Mux1/1 -> Road/1
  Demux1/9 -> Mux1/12
  ground4/1 -> Mux1/15
  ground3/1 -> Mux1/14
  gain/1 -> Multiply/2
  Demux1/1 -> Mux1/4
  surface friction in longitudinall direction/1 -> Mux1/19

== system Full_Car_Model/PLANT MODEL WITH MF-SWIFT/REAR RIGHT WHEEL/Subsystem2 ==
  speed : Inport
  Bus Selector : BusSelector  OutputSignals=States.x_u_dot_R_R,States.z_u_dot_R_R
  Constant : Constant  Value=0
  Mux : Mux  Inputs=3
  Velocity : Outport  VectorParamsAs1DForOutWhenUnconnected=off
  wires:
  Bus Selector/1 -> Mux/1  "<x_u_dot_R_R>"
  Constant/1 -> Mux/2  "No lateral component"
  Mux/1 -> Velocity/1
  speed/1 -> Bus Selector/1
  Bus Selector/2 -> Mux/3  "<z_u_dot_R_R>"

== system Full_Car_Model/PLANT MODEL WITH MF-SWIFT/REAR RIGHT WHEEL/Subsystem5 ==
  Angular Speed : Inport
  Constant1 : Constant  Value=0
  Constant2 : Constant  Value=0
  Constant3 : Constant  Value=0
  Mux : Mux  Inputs=3
  Terminator : Terminator
  AngularVelocity : Outport  VectorParamsAs1DForOutWhenUnconnected=off
  wires:
  Constant3/1 -> Mux/2
  Mux/1 -> AngularVelocity/1
  Angular Speed/1 -> Terminator/1
  Constant2/1 -> Mux/1
  Constant1/1 -> Mux/3

== system Full_Car_Model/PLANT MODEL WITH MF-SWIFT/REAR RIGHT WHEEL/Subsystem7 ==
  time : Inport
  gain : Inport  Port=2
  Demux1 : Demux  Outputs=9
  Multiply : Product  Inputs=**
  Mux1 : Mux  Inputs=20
  Step : Step  Time=1.216  After=0.02  SampleTime=0
  Terminator : Terminator
  ground{,1..7} (8 alike) : Ground
  rotation matrix1 : Constant  Value=[1 0 0 0 1 0 0 0 1]
  surface friction in lateral direction : Constant
  surface friction in longitudinall direction : Constant
  Road : Outport  VectorParamsAs1DForOutWhenUnconnected=off
  wires:
  Demux1/1 -> Mux1/4
  gain/1 -> Multiply/2
  ground3/1 -> Mux1/14
  ground4/1 -> Mux1/15
  Demux1/9 -> Mux1/12
  Mux1/1 -> Road/1
  ground5/1 -> Mux1/16
  Demux1/6 -> Mux1/9
  ground/1 -> Mux1/1
  Demux1/8 -> Mux1/11
  Demux1/7 -> Mux1/10
  Step/1 -> Multiply/1
  ground1/1 -> Mux1/2
  Demux1/3 -> Mux1/6
  ground6/1 -> Mux1/17
  ground7/1 -> Mux1/18
  Demux1/2 -> Mux1/5
  ground2/1 -> Mux1/13
  surface friction in lateral direction/1 -> Mux1/20
  surface friction in longitudinall direction/1 -> Mux1/19
  rotation matrix1/1 -> Demux1/1
  Demux1/5 -> Mux1/8
  Multiply/1 -> Mux1/3
  Demux1/4 -> Mux1/7
  time/1 -> Terminator/1

== system Full_Car_Model/PLANT MODEL WITH MF-SWIFT/SUSPENSION MODEL/LONGITUDINAL DYNAMICS ==
  States : Inport
  Forces : Inport  Port=2
  Bus Creator2 : BusCreator  Inputs=15
  Bus Selector4 : BusSelector  OutputSignals=Fk_x_R_L,Fc_x_R_L,Fk_x_R_R,Fc_x_R_R,Fk_x_F_L,Fc_x_F_L,Fk_x_F_R,Fc_x_F_R,F_x_R_L,F_x_R_R,F_x_F_L,F_x_F_R
  Bus Selector5 : BusSelector  OutputSignals=Longitudinal.x_b_dot
  Integrator1 : Integrator  InitialCondition=x_u_dot_ini_F_L
  Integrator12 : Integrator  InitialCondition=x_u_dot_ini_R_R
  Integrator13 : Integrator  InitialCondition=x_u_ini_R_R
  Integrator2 : Integrator  InitialCondition=x_u_ini_F_L
  Integrator3 : Integrator  InitialCondition=x_u_dot_ini_F_R
  Integrator4 : Integrator  InitialCondition=x_b_dot_ini
  Integrator5 : Integrator  InitialCondition=x_b_ini
  Integrator6 : Integrator  InitialCondition=x_u_dot_ini_R_L
  Integrator7 : Integrator  InitialCondition=x_u_ini_R_L
  Integrator8 : Integrator  InitialCondition=x_u_ini_F_R
  Longitudinal Balance : MATLAB Function  TreatAsAtomicUnit=on
  Longitudinal : Outport
  x_b_ddot : Outport  Port=2
  x_b_dot : Outport  Port=3
  x_b : Outport  Port=4
  x_u_ddot_R_L : Outport  Port=5
  x_u_dot_R_L : Outport  Port=6
  x_u_R_L : Outport  Port=7
  x_u_ddot_R_R : Outport  Port=8
  x_u_dot_R_R : Outport  Port=9
  x_u_R_R : Outport  Port=10
  x_u_ddot_F_L : Outport  Port=11
  x_u_dot_F_L : Outport  Port=12
  x_u_F_L : Outport  Port=13
  x_u_ddot_F_R : Outport  Port=14
  x_u_dot_F_R : Outport  Port=15
  x_u_F_R : Outport  Port=16
  wires:
  Integrator12/1 -> Integrator13/1, x_u_dot_R_R/1, Bus Creator2/8  "x_u_dot_R_R"
  Integrator5/1 -> x_b/1, Bus Creator2/1  "x_b"
  Integrator6/1 -> Integrator7/1, x_u_dot_R_L/1, Bus Creator2/5  "x_u_dot_R_L"
  Integrator7/1 -> x_u_R_L/1, Bus Creator2/4  "x_u_R_L"
  Longitudinal Balance/1(x_b_dot_dot) -> x_b_ddot/1, Integrator4/1, Bus Creator2/3  "x_b_ddot"
  Integrator1/1 -> Integrator2/1, x_u_dot_F_L/1, Bus Creator2/11  "x_u_dot_F_L"
  Integrator13/1 -> x_u_R_R/1, Bus Creator2/7  "x_u_R_R"
  Longitudinal Balance/3(x_u_dot_dot_R_R) -> Integrator12/1, x_u_ddot_R_R/1, Bus Creator2/9  "x_u_ddot_R_R"
  Integrator3/1 -> x_u_dot_F_R/1, Integrator8/1, Bus Creator2/14  "x_u_dot_F_R"
  Integrator8/1 -> x_u_F_R/1, Bus Creator2/13  "x_u_F_R"
  Integrator2/1 -> x_u_F_L/1, Bus Creator2/10  "x_u_F_L"
  Longitudinal Balance/4(x_u_dot_dot_F_L) -> Integrator1/1, x_u_ddot_F_L/1, Bus Creator2/12  "x_u_ddot_F_L"
  Longitudinal Balance/2(x_u_dot_dot_R_L) -> Integrator6/1, x_u_ddot_R_L/1, Bus Creator2/6  "x_u_ddot_R_L"
  Longitudinal Balance/5(x_u_dot_dot_F_R) -> x_u_ddot_F_R/1, Integrator3/1, Bus Creator2/15  "x_u_ddot_F_R"
  Bus Selector4/12 -> Longitudinal Balance/13(F_x_F_R)  "<F_x_F_R>"
  Bus Selector4/11 -> Longitudinal Balance/12(F_x_F_L)  "<F_x_F_L>"
  Bus Selector4/10 -> Longitudinal Balance/11(F_x_R_R)  "<F_x_R_R>"
  Bus Selector4/9 -> Longitudinal Balance/10(F_x_R_L)  "<F_x_R_L>"
  Bus Selector4/8 -> Longitudinal Balance/9(Fc_x_F_R)  "<Fc_x_F_R>"
  Bus Selector4/7 -> Longitudinal Balance/8(Fk_x_F_R)  "<Fk_x_F_R>"
  States/1 -> Bus Selector5/1
  Bus Selector5/1 -> Longitudinal Balance/1(x_b_dot)  "<x_b_dot>"
  Bus Selector4/2 -> Longitudinal Balance/3(Fc_x_R_L)  "<Fc_x_R_L>"
  Bus Selector4/5 -> Longitudinal Balance/6(Fk_x_F_L)  "<Fk_x_F_L>"
  Bus Selector4/4 -> Longitudinal Balance/5(Fc_x_R_R)  "<Fc_x_R_R>"
  Bus Selector4/3 -> Longitudinal Balance/4(Fk_x_R_R)  "<Fk_x_R_R>"
  Bus Selector4/6 -> Longitudinal Balance/7(Fc_x_F_L)  "<Fc_x_F_L>"
  Forces/1 -> Bus Selector4/1
  Bus Creator2/1 -> Longitudinal/1  "Longitudinal"
  Bus Selector4/1 -> Longitudinal Balance/2(Fk_x_R_L)  "<Fk_x_R_L>"
  Integrator4/1 -> Bus Creator2/2, x_b_dot/1, Integrator5/1  "x_b_dot"

== system Full_Car_Model/PLANT MODEL WITH MF-SWIFT/SUSPENSION MODEL/ROTATIONAL DYNAMICS ==
  Forces : Inport
  ACTIVE SUSPENSION_F_L : Constant  Value=0
  ACTIVE SUSPENSION_F_R : Constant  Value=0
  ACTIVE SUSPENSION_R_L : Constant  Value=0
  ACTIVE SUSPENSION_R_R : Constant  Value=0
  Angular balance : MATLAB Function  TreatAsAtomicUnit=on
  Bus Creator4 : BusCreator  Inputs=3
  Bus Selector2 : BusSelector  OutputSignals=Fk_x_R_L,Fc_x_R_L,Fk_z_R_L,Fc_z_R_L,Fk_x_R_R,Fc_x_R_R,Fk_z_R_R,Fc_z_R_R,Fk_x_F_L,Fc_x_F_L,Fk_z_F_L,Fc_z_F_L,Fk_x_F_R,Fc_x_F_R,Fk_z_F_R,Fc_z_F_R,Mz_AP
  Integrator16 : Integrator  InitialCondition=Pitch_dot
  Integrator17 : Integrator  InitialCondition=Pitch
  Rotational : Outport
  pitch_ddot : Outport  Port=2
  pitch_dot : Outport  Port=3
  pitch : Outport  Port=4
  wires:
  ACTIVE SUSPENSION_F_L/1 -> Angular balance/20(Fu_z_F_L)
  ACTIVE SUSPENSION_F_R/1 -> Angular balance/21(Fu_z_F_R)
  ACTIVE SUSPENSION_R_L/1 -> Angular balance/18(Fu_z_R_L)
  ACTIVE SUSPENSION_R_R/1 -> Angular balance/19(Fu_z_R_R)
  Integrator17/1 -> pitch/1, Bus Creator4/1  "pitch"
  Integrator16/1 -> Bus Creator4/2, pitch_dot/1, Integrator17/1  "pitch_dot"
  Bus Creator4/1 -> Rotational/1  "Rotational"
  Angular balance/1(pitch_dot_dot) -> pitch_ddot/1, Integrator16/1, Bus Creator4/3  "pitch_ddot"
  Forces/1 -> Bus Selector2/1
  Bus Selector2/1 -> Angular balance/1(Fk_x_R_L)  "<Fk_x_R_L>"
  Bus Selector2/2 -> Angular balance/2(Fc_x_R_L)  "<Fc_x_R_L>"
  Bus Selector2/3 -> Angular balance/3(Fk_z_R_L)  "<Fk_z_R_L>"
  Bus Selector2/4 -> Angular balance/4(Fc_z_R_L)  "<Fc_z_R_L>"
  Bus Selector2/5 -> Angular balance/5(Fk_x_R_R)  "<Fk_x_R_R>"
  Bus Selector2/6 -> Angular balance/6(Fc_x_R_R)  "<Fc_x_R_R>"
  Bus Selector2/7 -> Angular balance/7(Fk_z_R_R)  "<Fk_z_R_R>"
  Bus Selector2/8 -> Angular balance/8(Fc_z_R_R)  "<Fc_z_R_R>"
  Bus Selector2/9 -> Angular balance/9(Fk_x_F_L)  "<Fk_x_F_L>"
  Bus Selector2/10 -> Angular balance/10(Fc_x_F_L)  "<Fc_x_F_L>"
  Bus Selector2/11 -> Angular balance/11(Fk_z_F_L)  "<Fk_z_F_L>"
  Bus Selector2/12 -> Angular balance/12(Fc_z_F_L)  "<Fc_z_F_L>"
  Bus Selector2/13 -> Angular balance/13(Fk_x_F_R)  "<Fk_x_F_R>"
  Bus Selector2/14 -> Angular balance/14(Fc_x_F_R)  "<Fc_x_F_R>"
  Bus Selector2/15 -> Angular balance/15(Fk_z_F_R)  "<Fk_z_F_R>"
  Bus Selector2/16 -> Angular balance/16(Fc_z_F_R)  "<Fc_z_F_R>"
  Bus Selector2/17 -> Angular balance/17(Mz_AP)  "<Mz_AP>"

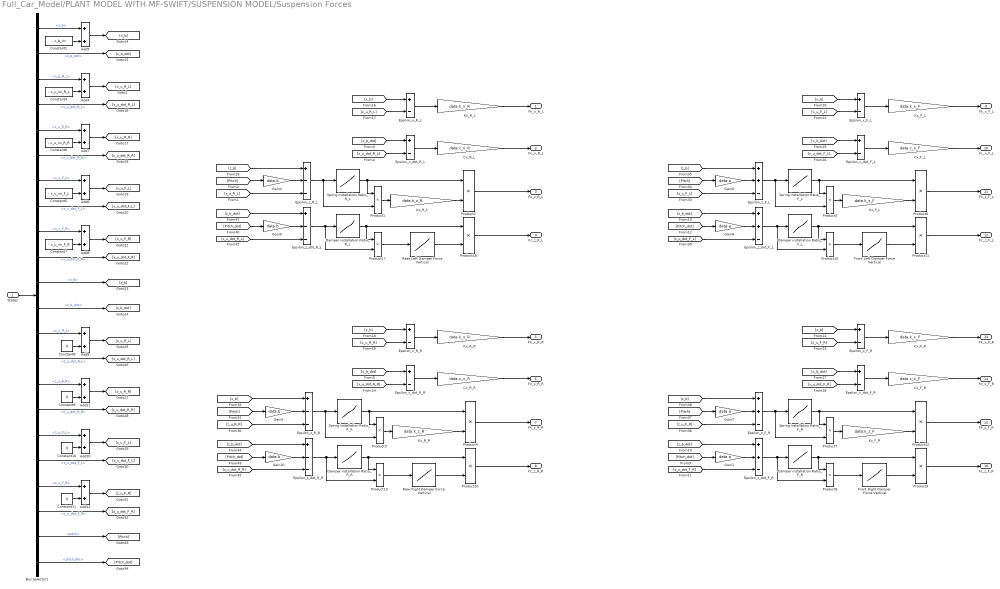
== system Full_Car_Model/PLANT MODEL WITH MF-SWIFT/SUSPENSION MODEL/Suspension Forces ==
  States : Inport
  Add{4..12} (9 alike) : Sum
  Bus Selector1 : BusSelector  OutputSignals=Longitudinal.x_b,Longitudinal.x_b_dot,Longitudinal.x_u_R_L,Longitudinal.x_u_dot_R_L,Longitudinal.x_u_R_R,Longitudinal.x_u_dot_R_R,Longitudinal.x_u_F_L,Longitudinal.x_u_dot_F_L,Longitudinal.x_u_F_R,Longitudinal.x_u_dot_F_R,Vertical.z_b,Vertical.z_b_dot,Vertical.z_u_R_L,Vertical.z_u_dot_R_L,Vertical.z_u_R_R,Vertical.z_u_dot_R_R,Vertical.z_u_F_L,Vertical.z_u_dot_F_L,Vertical.z_u_F_R,Vertical.z_u_dot_F_R,Rotational.pitch,Rotational.pitch_dot
  Constant{8..11} (4 alike) : Constant  Value=0
  Constant2 : Constant  Value=- x_b_ini
  Constant4 : Constant  Value=- x_u_ini_R_L
  Constant5 : Constant  Value=- x_u_ini_F_L
  Constant6 : Constant  Value=- x_u_ini_R_R
  Constant7 : Constant  Value=- x_u_ini_F_R
  Cx_F_L : Gain  Gain=data.c_x_F
  Cx_F_R : Gain  Gain=data.c_x_F
  Cx_R_L : Gain  Gain=data.c_x_R
  Cx_R_R : Gain  Gain=data.c_x_R
  Damper installation Ratio_F_L : Lookup_n-D  NumberOfTableDimensions=1  BreakpointsForDimension1=data.Wheel_displacement  Table=data.Damper_displacement./data.Wheel_displacement  InternalRulePriority=Speed  RndMeth=Simplest
  Damper installation Ratio_F_R : Lookup_n-D  NumberOfTableDimensions=1  BreakpointsForDimension1=data.Wheel_displacement  Table=data.Damper_displacement./data.Wheel_displacement  InternalRulePriority=Speed  RndMeth=Simplest
  Damper installation Ratio_R_L : Lookup_n-D  NumberOfTableDimensions=1  BreakpointsForDimension1=data.Wheel_displacement  Table=data.Damper_displacement./data.Wheel_displacement  InternalRulePriority=Speed  RndMeth=Simplest
  Damper installation Ratio_R_R : Lookup_n-D  NumberOfTableDimensions=1  BreakpointsForDimension1=data.Wheel_displacement  Table=data.Damper_displacement./data.Wheel_displacement  InternalRulePriority=Speed  RndMeth=Simplest
  Epsilon_x_F_L : Sum  Inputs=+-
  Epsilon_x_F_R : Sum  Inputs=+-
  Epsilon_x_R_L : Sum  Inputs=+-
  Epsilon_x_R_R : Sum  Inputs=+-
  Epsilon_x_dot_F_L : Sum  Inputs=+-
  Epsilon_x_dot_F_R : Sum  Inputs=+-
  Epsilon_x_dot_R_L : Sum  Inputs=+-
  Epsilon_x_dot_R_R : Sum  Inputs=+-
  Epsilon_z_F_L : Sum  Inputs=++-
  Epsilon_z_F_R : Sum  Inputs=++-
  Epsilon_z_R_L : Sum  Inputs=+--
  Epsilon_z_R_R : Sum  Inputs=+--
  Epsilon_z_dot_F_L : Sum  Inputs=++-
  Epsilon_z_dot_F_R : Sum  Inputs=++-
  Epsilon_z_dot_R_L : Sum  Inputs=+--
  Epsilon_z_dot_R_R : Sum  Inputs=+--
  Front Left Damper Force Vertical : Lookup_n-D  NumberOfTableDimensions=1  BreakpointsForDimension1=data.Damper_speed  Table=data.Damper_force_F  InternalRulePriority=Speed  RndMeth=Simplest
  Front Right Damper Force Vertical : Lookup_n-D  NumberOfTableDimensions=1  BreakpointsForDimension1=data.Damper_speed  Table=data.Damper_force_F  InternalRulePriority=Speed  RndMeth=Simplest
  Gain{1,6..8} (4 alike) : Gain  Gain=data.a
  Gain{4..5,9..10} (4 alike) : Gain  Gain=data.b
  Kx_F_L : Gain  Gain=data.k_x_F
  Kx_F_R : Gain  Gain=data.k_x_F
  Kx_R_L : Gain  Gain=data.k_x_R
  Kx_R_R : Gain  Gain=data.k_x_R
  Kz_F_L : Gain  Gain=data.k_z_F
  Kz_F_R : Gain  Gain=data.k_z_F
  Kz_R_L : Gain  Gain=data.k_z_R
  Kz_R_R : Gain  Gain=data.k_z_R
  Product{1..12,17..20} (16 alike) : Product
  Rear Left Damper Force Vertical : Lookup_n-D  NumberOfTableDimensions=1  BreakpointsForDimension1=data.Damper_speed  Table=data.Damper_force_R  InternalRulePriority=Speed  RndMeth=Simplest
  Rear Right Damper Force Vertical : Lookup_n-D  NumberOfTableDimensions=1  BreakpointsForDimension1=data.Damper_speed  Table=data.Damper_force_R  InternalRulePriority=Speed  RndMeth=Simplest
  Spring installation Ratio_F_L : Lookup_n-D  NumberOfTableDimensions=1  BreakpointsForDimension1=data.Wheel_displacement  Table=data.Spring_displacement./data.Wheel_displacement  InternalRulePriority=Speed  RndMeth=Simplest
  Spring installation Ratio_F_R : Lookup_n-D  NumberOfTableDimensions=1  BreakpointsForDimension1=data.Wheel_displacement  Table=data.Spring_displacement./data.Wheel_displacement  InternalRulePriority=Speed  RndMeth=Simplest
  Spring installation Ratio_R_L : Lookup_n-D  NumberOfTableDimensions=1  BreakpointsForDimension1=data.Wheel_displacement  Table=data.Spring_displacement./data.Wheel_displacement  InternalRulePriority=Speed  RndMeth=Simplest
  Spring installation Ratio_R_R : Lookup_n-D  NumberOfTableDimensions=1  BreakpointsForDimension1=data.Wheel_displacement  Table=data.Spring_displacement./data.Wheel_displacement  InternalRulePriority=Speed  RndMeth=Simplest
  Fk_x_R_L : Outport
  Fc_x_R_L : Outport  Port=2
  Fk_z_R_L : Outport  Port=3
  Fc_z_R_L : Outport  Port=4
  Fk_x_R_R : Outport  Port=5
  Fc_x_R_R : Outport  Port=6
  Fk_z_R_R : Outport  Port=7
  Fc_z_R_R : Outport  Port=8
  Fk_x_F_L : Outport  Port=9
  Fc_x_F_L : Outport  Port=10
  Fk_z_F_L : Outport  Port=11
  Fc_z_F_L : Outport  Port=12
  Fk_x_F_R : Outport  Port=13
  Fc_x_F_R : Outport  Port=14
  Fk_z_F_R : Outport  Port=15
  Fc_z_F_R : Outport  Port=16
  wires:
  Bus Selector1/22 -> [Pitch_dot]  "<pitch_dot>"
  Bus Selector1/21 -> [Pitch]  "<pitch>"
  Bus Selector1/13 -> Add9/1  "<z_u_R_L>"
  Constant8/1 -> Add9/2
  Add9/1 -> [z_u_R_L]
  Bus Selector1/15 -> Add11/1  "<z_u_R_R>"
  Constant9/1 -> Add11/2
  Add11/1 -> [z_u_R_R]
  Bus Selector1/14 -> [z_u_dot_R_L]  "<z_u_dot_R_L>"
  Bus Selector1/16 -> [z_u_dot_R_R]  "<z_u_dot_R_R>"
  Bus Selector1/18 -> [z_u_dot_F_L]  "<z_u_dot_F_L>"
  Add10/1 -> [z_u_F_L]
  Constant10/1 -> Add10/2
  Bus Selector1/17 -> Add10/1  "<z_u_F_L>"
  Bus Selector1/19 -> Add12/1  "<z_u_F_R>"
  Constant11/1 -> Add12/2
  Add12/1 -> [z_u_F_R]
  Bus Selector1/20 -> [z_u_dot_F_R]  "<z_u_dot_F_R>"
  Bus Selector1/12 -> [z_b_dot]  "<z_b_dot>"
  Bus Selector1/11 -> [z_b]  "<z_b>"
  Bus Selector1/10 -> [x_u_dot_F_R]  "<x_u_dot_F_R>"
  Add8/1 -> [x_u_F_R]
  Constant7/1 -> Add8/2
  Bus Selector1/9 -> Add8/1  "<x_u_F_R>"
  Bus Selector1/7 -> Add6/1  "<x_u_F_L>"
  Constant5/1 -> Add6/2
  Add6/1 -> [x_u_F_L]
  Bus Selector1/8 -> [x_u_dot_F_L]  "<x_u_dot_F_L>"
  Bus Selector1/6 -> [x_u_dot_R_R]  "<x_u_dot_R_R>"
  Bus Selector1/4 -> [x_u_dot_R_L]  "<x_u_dot_R_L>"
  Add7/1 -> [x_u_R_R]
  Constant6/1 -> Add7/2
  Bus Selector1/5 -> Add7/1  "<x_u_R_R>"
  Add4/1 -> [x_u_R_L]
  Constant4/1 -> Add4/2
  Bus Selector1/3 -> Add4/1  "<x_u_R_L>"
  Bus Selector1/2 -> [x_b_dot]  "<x_b_dot>"
  Add5/1 -> [x_b]
  Constant2/1 -> Add5/2
  Bus Selector1/1 -> Add5/1  "<x_b>"
  Epsilon_z_dot_R_R/1 -> Product19/2, Damper installation Ratio_R_R/1
  Product20/1 -> Fc_z_R_R/1
  Gain10/1 -> Epsilon_z_dot_R_R/2
  [z_b_dot] -> Epsilon_z_dot_R_R/1
  [Pitch_dot] -> Gain10/1
  [z_u_dot_R_R] -> Epsilon_z_dot_R_R/3
  Product19/1 -> Rear Right Damper Force Vertical/1
  Damper installation Ratio_R_R/1 -> Product19/1, Product20/1
  Rear Right Damper Force Vertical/1 -> Product20/2
  [z_b_dot] -> Epsilon_z_dot_R_L/1
  [z_u_dot_R_L] -> Epsilon_z_dot_R_L/3
  Epsilon_z_dot_R_L/1 -> Product17/2, Damper installation Ratio_R_L/1
  Gain9/1 -> Epsilon_z_dot_R_L/2
  Rear Left Damper Force Vertical/1 -> Product18/2
  [Pitch_dot] -> Gain9/1
  Damper installation Ratio_R_L/1 -> Product17/1, Product18/1
  Product17/1 -> Rear Left Damper Force Vertical/1
  Product18/1 -> Fc_z_R_L/1
  Product10/1 -> Front Left Damper Force Vertical/1
  Product11/1 -> Fc_z_F_L/1
  Damper installation Ratio_F_L/1 -> Product10/1, Product11/1
  [Pitch_dot] -> Gain8/1
  [z_u_dot_F_L] -> Epsilon_z_dot_F_L/3
  [z_b_dot] -> Epsilon_z_dot_F_L/1
  Front Left Damper Force Vertical/1 -> Product11/2
  Epsilon_z_dot_F_L/1 -> Damper installation Ratio_F_L/1, Product10/2
  Gain8/1 -> Epsilon_z_dot_F_L/2
  Product8/1 -> Front Right Damper Force Vertical/1
  Product9/1 -> Fc_z_F_R/1
  Damper installation Ratio_F_R/1 -> Product8/1, Product9/1
  [Pitch_dot] -> Gain1/1
  [z_u_dot_F_R] -> Epsilon_z_dot_F_R/3
  [z_b_dot] -> Epsilon_z_dot_F_R/1
  Front Right Damper Force Vertical/1 -> Product9/2
  Epsilon_z_dot_F_R/1 -> Damper installation Ratio_F_R/1, Product8/2
  Gain1/1 -> Epsilon_z_dot_F_R/2
  Product12/1 -> Fk_z_F_R/1
  Spring installation Ratio_F_R/1 -> Product12/1, Product7/1
  Epsilon_z_F_R/1 -> Spring installation Ratio_F_R/1, Product7/2
  [Pitch] -> Gain7/1
  [z_u_F_R] -> Epsilon_z_F_R/3
  Kz_F_R/1 -> Product12/2
  [z_b] -> Epsilon_z_F_R/1
  Product7/1 -> Kz_F_R/1
  Gain7/1 -> Epsilon_z_F_R/2
  Gain6/1 -> Epsilon_z_F_L/2
  Product5/1 -> Kz_F_L/1
  [z_b] -> Epsilon_z_F_L/1
  Kz_F_L/1 -> Product6/2
  [z_u_F_L] -> Epsilon_z_F_L/3
  [Pitch] -> Gain6/1
  Epsilon_z_F_L/1 -> Product5/2, Spring installation Ratio_F_L/1
  Spring installation Ratio_F_L/1 -> Product5/1, Product6/1
  Product6/1 -> Fk_z_F_L/1
  Product4/1 -> Fk_z_R_R/1
  Spring installation Ratio_R_R/1 -> Product3/1, Product4/1
  Epsilon_z_R_R/1 -> Product3/2, Spring installation Ratio_R_R/1
  [Pitch] -> Gain5/1
  Product3/1 -> Kz_R_R/1
  [z_u_R_R] -> Epsilon_z_R_R/3
  Gain5/1 -> Epsilon_z_R_R/2
  Kz_R_R/1 -> Product4/2
  [z_b] -> Epsilon_z_R_R/1
  [z_u_R_L] -> Epsilon_z_R_L/3
  Spring installation Ratio_R_L/1 -> Product1/1, Product2/1
  Product1/1 -> Kz_R_L/1
  [Pitch] -> Gain4/1
  Epsilon_z_R_L/1 -> Product1/2, Spring installation Ratio_R_L/1
  Gain4/1 -> Epsilon_z_R_L/2
  [z_b] -> Epsilon_z_R_L/1
  Product2/1 -> Fk_z_R_L/1
  Kz_R_L/1 -> Product2/2
  Epsilon_x_dot_F_R/1 -> Cx_F_R/1
  [x_u_dot_F_R] -> Epsilon_x_dot_F_R/2
  [x_b_dot] -> Epsilon_x_dot_F_R/1
  [x_b_dot] -> Epsilon_x_dot_F_L/1
  [x_u_dot_F_L] -> Epsilon_x_dot_F_L/2
  Epsilon_x_dot_F_L/1 -> Cx_F_L/1
  Cx_F_R/1 -> Fc_x_F_R/1
  Cx_F_L/1 -> Fc_x_F_L/1
  Cx_R_R/1 -> Fc_x_R_R/1
  Epsilon_x_dot_R_R/1 -> Cx_R_R/1
  [x_b_dot] -> Epsilon_x_dot_R_R/1
  [x_u_dot_R_R] -> Epsilon_x_dot_R_R/2
  Epsilon_x_dot_R_L/1 -> Cx_R_L/1
  [x_u_dot_R_L] -> Epsilon_x_dot_R_L/2
  [x_b_dot] -> Epsilon_x_dot_R_L/1
  Cx_R_L/1 -> Fc_x_R_L/1
  [x_b] -> Epsilon_x_F_R/1
  [x_u_F_R] -> Epsilon_x_F_R/2
  Epsilon_x_F_R/1 -> Kx_F_R/1
  [x_u_F_L] -> Epsilon_x_F_L/2
  Epsilon_x_F_L/1 -> Kx_F_L/1
  [x_b] -> Epsilon_x_F_L/1
  [x_u_R_R] -> Epsilon_x_R_R/2
  Epsilon_x_R_R/1 -> Kx_R_R/1
  [x_b] -> Epsilon_x_R_R/1
  Epsilon_x_R_L/1 -> Kx_R_L/1
  [x_u_R_L] -> Epsilon_x_R_L/2
  [x_b] -> Epsilon_x_R_L/1
  Kx_R_R/1 -> Fk_x_R_R/1
  Kx_F_R/1 -> Fk_x_F_R/1
  Kx_R_L/1 -> Fk_x_R_L/1
  Kx_F_L/1 -> Fk_x_F_L/1
  States/1 -> Bus Selector1/1

== system Full_Car_Model/PLANT MODEL WITH MF-SWIFT/SUSPENSION MODEL/VERTICAL DYNAMICS ==
  Forces : Inport
  ACTIVE SUSPENSION_F_L : Constant  Value=0
  ACTIVE SUSPENSION_F_R : Constant  Value=0
  ACTIVE SUSPENSION_R_L : Constant  Value=0
  ACTIVE SUSPENSION_R_R : Constant  Value=0
  Bus Creator : BusCreator  Inputs=15
  Bus Selector1 : BusSelector  OutputSignals=Fk_z_R_L,Fc_z_R_L,Fk_z_R_R,Fc_z_R_R,Fk_z_F_L,Fc_z_F_L,Fk_z_F_R,Fc_z_F_R,F_z_R_L,F_z_R_R,F_z_F_L,F_z_F_R,Fu_AP_F,Fu_AP_R,Fz_AP
  Integrator1 : Integrator  InitialCondition=z_u_dot_ini_F_L
  Integrator12 : Integrator  InitialCondition=z_u_dot_ini_R_R
  Integrator13 : Integrator  InitialCondition=z_u_ini_R_R
  Integrator2 : Integrator  InitialCondition=z_u_ini_F_L
  Integrator3 : Integrator  InitialCondition=z_u_dot_ini_F_R
  Integrator4 : Integrator  InitialCondition=z_b_dot_ini
  Integrator5 : Integrator  InitialCondition=z_b_ini
  Integrator6 : Integrator  InitialCondition=z_u_dot_ini_R_L
  Integrator7 : Integrator  InitialCondition=z_u_ini_R_L
  Integrator8 : Integrator  InitialCondition=z_u_ini_F_R
  Vertical Balance : MATLAB Function  TreatAsAtomicUnit=on
  Vertical : Outport
  z_b_ddot : Outport  Port=2
  z_b_dot : Outport  Port=3
  z_b : Outport  Port=4
  z_u_ddot_R_L : Outport  Port=5
  z_u_dot_R_L : Outport  Port=6
  z_u_R_L : Outport  Port=7
  z_u_ddot_R_R : Outport  Port=8
  z_u_dot_R_R : Outport  Port=9
  z_u_R_R : Outport  Port=10
  z_u_ddot_F_L : Outport  Port=11
  z_u_dot_F_L : Outport  Port=12
  z_u_F_L : Outport  Port=13
  z_u_ddot_F_R : Outport  Port=14
  z_u_dot_F_R : Outport  Port=15
  z_u_F_R : Outport  Port=16
  wires:
  Bus Selector1/15 -> Vertical Balance/15(Fz_AP)  "<Fz_AP>"
  Bus Selector1/14 -> Vertical Balance/14(Fu_AP_R)  "<Fu_AP_R>"
  Bus Selector1/13 -> Vertical Balance/13(Fu_AP_F)  "<Fu_AP_F>"
  ACTIVE SUSPENSION_F_L/1 -> Vertical Balance/18(Fu_z_F_L)
  ACTIVE SUSPENSION_F_R/1 -> Vertical Balance/19(Fu_z_F_R)
  Vertical Balance/5(z_u_dot_dot_F_R) -> Integrator3/1, z_u_ddot_F_R/1, Bus Creator/15  "z_u_ddot_F_R"
  Integrator8/1 -> z_u_F_R/1, Bus Creator/13  "z_u_F_R"
  Integrator3/1 -> z_u_dot_F_R/1, Integrator8/1, Bus Creator/14  "z_u_dot_F_R"
  Integrator1/1 -> z_u_dot_F_L/1, Integrator2/1, Bus Creator/11  "z_u_dot_F_L"
  Integrator2/1 -> z_u_F_L/1, Bus Creator/10  "z_u_F_L"
  Vertical Balance/4(z_u_dot_dot_F_L) -> Integrator1/1, z_u_ddot_F_L/1, Bus Creator/12  "z_u_ddot_F_L"
  Bus Selector1/1 -> Vertical Balance/1(Fk_z_R_L)  "<Fk_z_R_L>"
  Bus Selector1/2 -> Vertical Balance/2(Fc_z_R_L)  "<Fc_z_R_L>"
  Bus Selector1/3 -> Vertical Balance/3(Fk_z_R_R)  "<Fk_z_R_R>"
  Bus Selector1/4 -> Vertical Balance/4(Fc_z_R_R)  "<Fc_z_R_R>"
  Bus Selector1/5 -> Vertical Balance/5(Fk_z_F_L)  "<Fk_z_F_L>"
  Bus Selector1/6 -> Vertical Balance/6(Fc_z_F_L)  "<Fc_z_F_L>"
  Bus Selector1/7 -> Vertical Balance/7(Fk_z_F_R)  "<Fk_z_F_R>"
  Bus Selector1/8 -> Vertical Balance/8(Fc_z_F_R)  "<Fc_z_F_R>"
  Bus Selector1/9 -> Vertical Balance/9(F_z_R_L)  "<F_z_R_L>"
  Bus Selector1/10 -> Vertical Balance/10(F_z_R_R)  "<F_z_R_R>"
  Bus Selector1/11 -> Vertical Balance/11(F_z_F_L)  "<F_z_F_L>"
  Bus Selector1/12 -> Vertical Balance/12(F_z_F_R)  "<F_z_F_R>"
  ACTIVE SUSPENSION_R_R/1 -> Vertical Balance/17(Fu_z_R_R)
  ACTIVE SUSPENSION_R_L/1 -> Vertical Balance/16(Fu_z_R_L)
  Vertical Balance/1(z_b_dot_dot) -> Bus Creator/3, z_b_ddot/1, Integrator4/1  "z_b_ddot"
  Integrator7/1 -> Bus Creator/4, z_u_R_L/1  "z_u_R_L"
  Integrator5/1 -> Bus Creator/1, z_b/1  "z_b"
  Bus Creator/1 -> Vertical/1  "Vertical"
  Integrator13/1 -> Bus Creator/7, z_u_R_R/1  "z_u_R_R"
  Vertical Balance/3(z_u_dot_dot_R_R) -> Integrator12/1, z_u_ddot_R_R/1, Bus Creator/9  "z_u_ddot_R_R"
  Integrator12/1 -> Integrator13/1, z_u_dot_R_R/1, Bus Creator/8  "z_u_dot_R_R"
  Integrator4/1 -> Integrator5/1, z_b_dot/1, Bus Creator/2  "z_b_dot"
  Forces/1 -> Bus Selector1/1
  Integrator6/1 -> Integrator7/1, Bus Creator/5, z_u_dot_R_L/1  "z_u_dot_R_L"
  Vertical Balance/2(z_u_dot_dot_R_L) -> Integrator6/1, z_u_ddot_R_L/1, Bus Creator/6  "z_u_ddot_R_L"

== matlab function Full_Car_Model/CONTROLLER REAR RIGHT/ROAD PREVIEW/NO_ROAD_PREVIEW ==
  data: w input; OnlineData output; Tm_req input; Tm_req_R2 input; Tm_req_F_L input; Tm_req_F_R input; N parameter; mu_act input; sigma_ref input
function OnlineData=OnlineDataArray(w, Tm_req, Tm_req_R2, Tm_req_F_L, Tm_req_F_R, N, mu_act, sigma_ref)

OnlineData = repmat([w; 0; Tm_req; Tm_req_R2; Tm_req_F_L; Tm_req_F_R; mu_act; sigma_ref],N+1,1);
end
